simulink model "gm_comm8qamtxrxhdl"  (R2025b)
settings: Solver=FixedStepDiscrete  StartTime=0.0  StopTime=20000*qam_params.symbolPeriod  RelTol=1e-3
PreLoadFcn:
  | qam_params = comm8qamtxrxhdl_init;
InitFcn:
  | qam_params = comm8qamtxrxhdl_init;
undefined symbols (not defined in the file or in its folder): Add, Shift
libraries: simulink x4, hdlsllib x4, dspsigops x2, commchan3 x1, commrflib2 x1, dsphdlmathfun2 x1, dsphdlsigops2 x1, dspmlti4 x1, simulink_need_slupdate x1, hdlmdlgenlib x1, commdigbbndam3 x1, commsequence2 x1
(part 3 of 3)

== system gm_comm8qamtxrxhdl/QAM Tx HDL/Data Generation & Packetization/Group Bits ==
  Bits In : Inport  OutDataTypeStr=boolean  PortDimensions=1  SampleTime=3.33333333333333e-07
  Bit Concat : hdlsllib/Logic and Bit Operations/Bit Concat  numInputs=3
  Delay : Delay  DelayLength=double(1)  InitialCondition=0  SampleTime=3.33333333333333e-07
  Delay4 : Delay  DelayLength=double(2)  InitialCondition=0  SampleTime=3.33333333333333e-07
  Delay5 : Delay  DelayLength=double(1)  InitialCondition=0  SampleTime=3.33333333333333e-07
  Downsample : DownSample  N=double(3)  phase=double(0)  RateOptions=Allow multirate processing  AllowArbitraryFixedInput=on
  Integer Out : Outport  SampleTime=1e-06  VectorParamsAs1DForOutWhenUnconnected=off
  wires:
  Delay/1 -> Downsample/1
  Bits In/1 -> Bit Concat/3, Delay4/1, Delay5/1
  Delay4/1 -> Bit Concat/1
  Downsample/1 -> Integer Out/1
  Delay5/1 -> Bit Concat/2
  Bit Concat/1 -> Delay/1

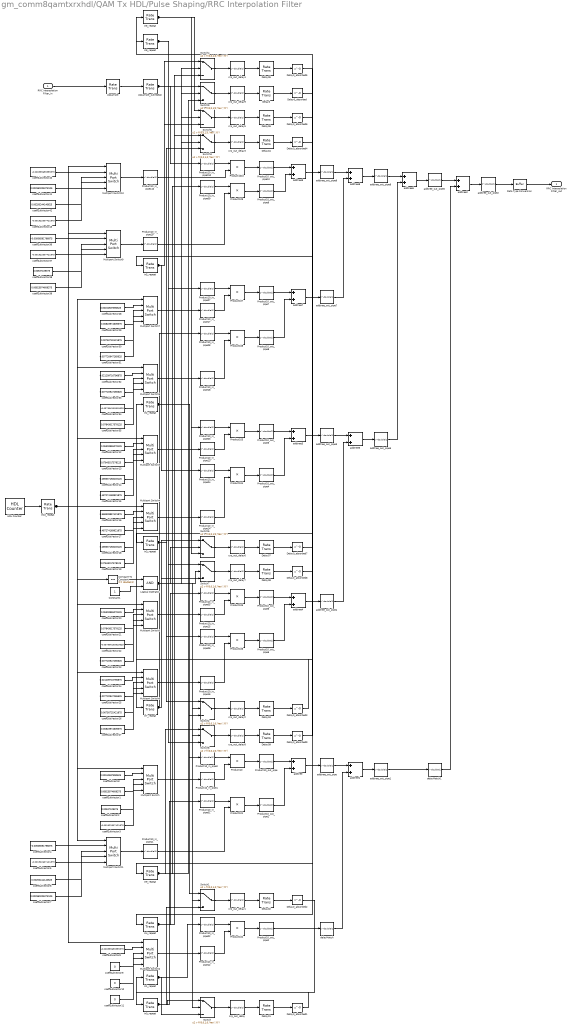
== system gm_comm8qamtxrxhdl/QAM Tx HDL/Pulse Shaping/RRC Interpolation Filter ==
  RRC Interpolation Filter_In : Inport  OutDataTypeStr=fixdt(1, 16, 15)  SampleTime=1e-06
      settings: SignalType=complex
  Compare To Constant : simulink/Logic and Bit Operations/Compare To Constant  relop===  const=double(3)  OutDataTypeStr=boolean
  Constant1 : Constant  OutDataTypeStr=fixdt(0, 1, 0)  SampleTime=8.33333333333333e-08
  Data Type Conversion : hdlmdlgenlib/Buffer
  Delay0 : RateTransition  InitialCondition=double(0)  OutPortSampleTimeOpt=Multiple of input port sample time  OutPortSampleTimeMultiple=3
  Delay01 : RateTransition  InitialCondition=double(0)  OutPortSampleTimeOpt=Multiple of input port sample time  OutPortSampleTimeMultiple=3
  Delay02 : RateTransition  InitialCondition=double(0)  OutPortSampleTimeOpt=Multiple of input port sample time  OutPortSampleTimeMultiple=3
  Delay03 : RateTransition  InitialCondition=double(0)  OutPortSampleTimeOpt=Multiple of input port sample time  OutPortSampleTimeMultiple=3
  Delay04 : RateTransition  InitialCondition=double(0)  OutPortSampleTimeOpt=Multiple of input port sample time  OutPortSampleTimeMultiple=3
  Delay05 : RateTransition  InitialCondition=double(0)  OutPortSampleTimeOpt=Multiple of input port sample time  OutPortSampleTimeMultiple=3
  Delay06 : RateTransition  InitialCondition=double(0)  OutPortSampleTimeOpt=Multiple of input port sample time  OutPortSampleTimeMultiple=3
  Delay07 : RateTransition  InitialCondition=double(0)  OutPortSampleTimeOpt=Multiple of input port sample time  OutPortSampleTimeMultiple=3
  Delay08 : RateTransition  InitialCondition=double(0)  OutPortSampleTimeOpt=Multiple of input port sample time  OutPortSampleTimeMultiple=3
  Delay09 : RateTransition  InitialCondition=double(0)  OutPortSampleTimeOpt=Multiple of input port sample time  OutPortSampleTimeMultiple=3
  Delay0_absorbed{,1..9} (10 alike) : Delay  DelayLength=0
  HDL Counter : hdlsllib/Sources/HDL Counter  CountType=Count limited  CountInit=double(0)  CountStep=double(1)  CountMax=double(3)  CountFromType=Initial value  CountFrom=double(0)  CountResetPort=off  CountLoadPort=off  CountEnbPort=off  CountDirPort=off  CountHitOutputPort=off  CountDataType=Unsigned  CountWordLen=2  CountFracLen=0  CountSampTime=2.5e-07
  Logical Operator : Logic  AllPortsSameDT=off  OutDataTypeStr=fixdt(0, 1, 0)  SampleTime=8.33333333333333e-08
  Multiport Switch{,1..10} (11 alike) : MultiPortSwitch  DataPortOrder=Zero-based contiguous  Inputs=4  DiagnosticForDefault=None  zeroidx=on  OutDataTypeStr=fixdt(1, 16, 15)  SampleTime=8.33333333333333e-08  SaturateOnIntegerOverflow=off  InputSameDT=off
  Product{10,101..109,1010} (11 alike) : Product  Inputs=**  OutDataTypeStr=fixdt(1, 16, 15)  RndMeth=Nearest  SaturateOnIntegerOverflow=on  SampleTime=8.33333333333333e-08
  Product10_in_pipe{0..1,11..19,110} (12 alike) : Delay  DelayLength=double(1)  InitialCondition=0  SampleTime=8.33333333333333e-08
  Product10_in_pipe01 : Delay  DelayLength=double(1)  InitialCondition=0  SampleTime=8.33333333333333e-08
  Product10_in_pipe010 : Delay  DelayLength=double(1)  InitialCondition=0  SampleTime=8.33333333333333e-08
  Product10_in_pipe02 : Delay  DelayLength=double(1)  InitialCondition=0  SampleTime=8.33333333333333e-08
  Product10_in_pipe03 : Delay  DelayLength=double(1)  InitialCondition=0  SampleTime=8.33333333333333e-08
  Product10_in_pipe04 : Delay  DelayLength=double(1)  InitialCondition=0  SampleTime=8.33333333333333e-08
  Product10_in_pipe05 : Delay  DelayLength=double(1)  InitialCondition=0  SampleTime=8.33333333333333e-08
  Product10_in_pipe06 : Delay  DelayLength=double(1)  InitialCondition=0  SampleTime=8.33333333333333e-08
  Product10_in_pipe07 : Delay  DelayLength=double(1)  InitialCondition=0  SampleTime=8.33333333333333e-08
  Product10_in_pipe08 : Delay  DelayLength=double(1)  InitialCondition=0  SampleTime=8.33333333333333e-08
  Product10_in_pipe09 : Delay  DelayLength=double(1)  InitialCondition=0  SampleTime=8.33333333333333e-08
  Product10_out_pipe{,1..10} (11 alike) : Delay  DelayLength=double(2)  InitialCondition=0  SampleTime=8.33333333333333e-08
  Switch{,1..9} (10 alike) : Switch  Criteria=u2 > Threshold  Threshold="fi(0,0,1,0,\"hex\",\"0\")"  OutDataTypeStr=fixdt(1, 16, 15)  SampleTime=8.33333333333333e-08  SaturateOnIntegerOverflow=off  InputSameDT=off
  Upsample : RateTransition  Integrity=off  Deterministic=off  OutPortSampleTimeOpt=Multiple of input port sample time  OutPortSampleTimeMultiple=1/4
  Upsample_outrepeat : RateTransition  Integrity=off  Deterministic=off  OutPortSampleTimeOpt=Multiple of input port sample time  OutPortSampleTimeMultiple=1/3
  addtree{,1..9} (10 alike) : Sum  OutDataTypeStr=fixdt(1, 16, 15)  RndMeth=Nearest  SaturateOnIntegerOverflow=on  SampleTime=8.33333333333333e-08
  addtree_out_pipe{,1..9} (10 alike) : Delay  DelayLength=double(1)  InitialCondition=0  SampleTime=8.33333333333333e-08
  coeffSubVector : Constant  Value=0.00152587890625  OutDataTypeStr=fixdt(1, 16, 15)  SampleTime=8.33333333333333e-08
  coeffSubVector1 : Constant  Value=0.00823974609375  OutDataTypeStr=fixdt(1, 16, 15)  SampleTime=8.33333333333333e-08
  coeffSubVector10 : Constant  Value=0  OutDataTypeStr=fixdt(1, 16, 15)  SampleTime=8.33333333333333e-08
  coeffSubVector11 : Constant  Value=0  OutDataTypeStr=fixdt(1, 16, 15)  SampleTime=8.33333333333333e-08
  coeffSubVector12 : Constant  Value=-0.05303955078125  OutDataTypeStr=fixdt(1, 16, 15)  SampleTime=8.33333333333333e-08
  coeffSubVector13 : Constant  Value=0.07843017578125  OutDataTypeStr=fixdt(1, 16, 15)  SampleTime=8.33333333333333e-08
  coeffSubVector14 : Constant  Value=0.289337158203125  OutDataTypeStr=fixdt(1, 16, 15)  SampleTime=8.33333333333333e-08
  coeffSubVector15 : Constant  Value=0.487274169921875  OutDataTypeStr=fixdt(1, 16, 15)  SampleTime=8.33333333333333e-08
  coeffSubVector16 : Constant  Value=0.568328857421875  OutDataTypeStr=fixdt(1, 16, 15)  SampleTime=8.33333333333333e-08
  coeffSubVector17 : Constant  Value=0.487274169921875  OutDataTypeStr=fixdt(1, 16, 15)  SampleTime=8.33333333333333e-08
  coeffSubVector18 : Constant  Value=0.289337158203125  OutDataTypeStr=fixdt(1, 16, 15)  SampleTime=8.33333333333333e-08
  coeffSubVector19 : Constant  Value=0.07843017578125  OutDataTypeStr=fixdt(1, 16, 15)  SampleTime=8.33333333333333e-08
  coeffSubVector2 : Constant  Value=0.00537109375  OutDataTypeStr=fixdt(1, 16, 15)  SampleTime=8.33333333333333e-08
  coeffSubVector20 : Constant  Value=-0.05303955078125  OutDataTypeStr=fixdt(1, 16, 15)  SampleTime=8.33333333333333e-08
  coeffSubVector21 : Constant  Value=-0.07843017578125  OutDataTypeStr=fixdt(1, 16, 15)  SampleTime=8.33333333333333e-08
  coeffSubVector22 : Constant  Value=-0.037506103515625  OutDataTypeStr=fixdt(1, 16, 15)  SampleTime=8.33333333333333e-08
  coeffSubVector{23,25,31,33} (4 alike) : Constant  Value=0.007720947265625  OutDataTypeStr=fixdt(1, 16, 15)  SampleTime=8.33333333333333e-08
  coeffSubVector24 : Constant  Value=0.021209716796875  OutDataTypeStr=fixdt(1, 16, 15)  SampleTime=8.33333333333333e-08
  coeffSubVector26 : Constant  Value=-0.00750732421875  OutDataTypeStr=fixdt(1, 16, 15)  SampleTime=8.33333333333333e-08
  coeffSubVector27 : Constant  Value=-0.00823974609375  OutDataTypeStr=fixdt(1, 16, 15)  SampleTime=8.33333333333333e-08
  coeffSubVector28 : Constant  Value=0.00152587890625  OutDataTypeStr=fixdt(1, 16, 15)  SampleTime=8.33333333333333e-08
  coeffSubVector29 : Constant  Value=-0.00823974609375  OutDataTypeStr=fixdt(1, 16, 15)  SampleTime=8.33333333333333e-08
  coeffSubVector{3,5,37,43} (4 alike) : Constant  Value=-0.001922607421875  OutDataTypeStr=fixdt(1, 16, 15)  SampleTime=8.33333333333333e-08
  coeffSubVector30 : Constant  Value=-0.00750732421875  OutDataTypeStr=fixdt(1, 16, 15)  SampleTime=8.33333333333333e-08
  coeffSubVector32 : Constant  Value=0.021209716796875  OutDataTypeStr=fixdt(1, 16, 15)  SampleTime=8.33333333333333e-08
  coeffSubVector34 : Constant  Value=-0.037506103515625  OutDataTypeStr=fixdt(1, 16, 15)  SampleTime=8.33333333333333e-08
  coeffSubVector35 : Constant  Value=-0.07843017578125  OutDataTypeStr=fixdt(1, 16, 15)  SampleTime=8.33333333333333e-08
  coeffSubVector36 : Constant  Value=-0.00506591796875  OutDataTypeStr=fixdt(1, 16, 15)  SampleTime=8.33333333333333e-08
  coeffSubVector38 : Constant  Value=0.00537109375  OutDataTypeStr=fixdt(1, 16, 15)  SampleTime=8.33333333333333e-08
  coeffSubVector39 : Constant  Value=0.00823974609375  OutDataTypeStr=fixdt(1, 16, 15)  SampleTime=8.33333333333333e-08
  coeffSubVector4 : Constant  Value=-0.00506591796875  OutDataTypeStr=fixdt(1, 16, 15)  SampleTime=8.33333333333333e-08
  coeffSubVector40 : Constant  Value=-0.000335693359375  OutDataTypeStr=fixdt(1, 16, 15)  SampleTime=8.33333333333333e-08
  coeffSubVector41 : Constant  Value=0.002960205078125  OutDataTypeStr=fixdt(1, 16, 15)  SampleTime=8.33333333333333e-08
  coeffSubVector42 : Constant  Value=0.00250244140625  OutDataTypeStr=fixdt(1, 16, 15)  SampleTime=8.33333333333333e-08
  coeffSubVector6 : Constant  Value=0.00250244140625  OutDataTypeStr=fixdt(1, 16, 15)  SampleTime=8.33333333333333e-08
  coeffSubVector7 : Constant  Value=0.002960205078125  OutDataTypeStr=fixdt(1, 16, 15)  SampleTime=8.33333333333333e-08
  coeffSubVector8 : Constant  Value=-0.000335693359375  OutDataTypeStr=fixdt(1, 16, 15)  SampleTime=8.33333333333333e-08
  coeffSubVector9 : Constant  Value=0  OutDataTypeStr=fixdt(1, 16, 15)  SampleTime=8.33333333333333e-08
  crp_out_delay{,1..9} (10 alike) : Delay  DelayLength=double(1)  InitialCondition=0  SampleTime=8.33333333333333e-08
  delayMatch : Delay  DelayLength=double(1)  InitialCondition=0  SampleTime=8.33333333333333e-08
  delayMatch1 : Delay  DelayLength=double(1)  InitialCondition=0  SampleTime=8.33333333333333e-08
  in0_repeat : RateTransition  Integrity=off  Deterministic=off  OutPortSampleTimeOpt=Multiple of input port sample time  OutPortSampleTimeMultiple=1/3
  in10_repeat : RateTransition  Integrity=off  Deterministic=off  OutPortSampleTimeOpt=Multiple of input port sample time  OutPortSampleTimeMultiple=1/3
  in1_repeat : RateTransition  Integrity=off  Deterministic=off  OutPortSampleTimeOpt=Multiple of input port sample time  OutPortSampleTimeMultiple=1/3
  in2_repeat : RateTransition  Integrity=off  Deterministic=off  OutPortSampleTimeOpt=Multiple of input port sample time  OutPortSampleTimeMultiple=1/3
  in3_repeat : RateTransition  Integrity=off  Deterministic=off  OutPortSampleTimeOpt=Multiple of input port sample time  OutPortSampleTimeMultiple=1/3
  in4_repeat : RateTransition  Integrity=off  Deterministic=off  OutPortSampleTimeOpt=Multiple of input port sample time  OutPortSampleTimeMultiple=1/3
  in5_repeat : RateTransition  Integrity=off  Deterministic=off  OutPortSampleTimeOpt=Multiple of input port sample time  OutPortSampleTimeMultiple=1/3
  in6_repeat : RateTransition  Integrity=off  Deterministic=off  OutPortSampleTimeOpt=Multiple of input port sample time  OutPortSampleTimeMultiple=1/3
  in7_repeat : RateTransition  Integrity=off  Deterministic=off  OutPortSampleTimeOpt=Multiple of input port sample time  OutPortSampleTimeMultiple=1/3
  in8_repeat : RateTransition  Integrity=off  Deterministic=off  OutPortSampleTimeOpt=Multiple of input port sample time  OutPortSampleTimeMultiple=1/3
  in9_repeat : RateTransition  Integrity=off  Deterministic=off  OutPortSampleTimeOpt=Multiple of input port sample time  OutPortSampleTimeMultiple=1/3
  RRC Interpolation Filter_out : Outport  OutDataTypeStr=fixdt(1, 16, 15)  SampleTime=8.33333333333333e-08
      settings: SignalType=complex
  wires:
  addtree_out_pipe1/1 -> delayMatch1/1
  coeffSubVector2/1 -> Multiport Switch/4
  Product10_in_pipe08/1 -> Product108/1
  addtree2/1 -> addtree_out_pipe2/1
  Switch/1 -> crp_out_delay/1
  addtree8/1 -> addtree_out_pipe8/1
  addtree_out_pipe9/1 -> addtree8/1
  Logical Operator/1 -> Switch/2, Switch1/2, Switch2/2, Switch4/2, Switch5/2, Switch6/2, Switch7/2, Switch9/2, Switch3/2, Switch8/2
  Product10_in_pipe010/1 -> Product1010/1
  addtree/1 -> addtree_out_pipe/1
  Product10_out_pipe3/1 -> addtree3/1
  addtree5/1 -> addtree_out_pipe5/1
  Delay09/1 -> Delay0_absorbed9/1
  Product10_in_pipe09/1 -> Product109/1
  Product10_in_pipe01/1 -> Product101/1
  coeffSubVector27/1 -> Multiport Switch6/5
  Product10_in_pipe18/1 -> Product108/2
  coeffSubVector24/1 -> Multiport Switch6/2
  Product10_in_pipe17/1 -> Product107/2
  addtree_out_pipe4/1 -> addtree5/2
  Multiport Switch9/1 -> Product10_in_pipe19/1
  Delay0_absorbed/1 -> in9_repeat/1
  Product108/1 -> Product10_out_pipe8/1
  addtree_out_pipe7/1 -> addtree8/2
  Product10_in_pipe07/1 -> Product107/1
  Delay0_absorbed1/1 -> in1_repeat/1
  coeffSubVector36/1 -> Multiport Switch9/2
  Product10_in_pipe16/1 -> Product106/2
  Product10_in_pipe03/1 -> Product103/1
  coeffSubVector40/1 -> Multiport Switch10/2
  Upsample/1 -> Upsample_outrepeat/1
  Multiport Switch4/1 -> Product10_in_pipe14/1
  Product10_in_pipe12/1 -> Product102/2
  addtree9/1 -> addtree_out_pipe9/1
  coeffSubVector21/1 -> Multiport Switch5/3
  Product10_in_pipe05/1 -> Product105/1
  Switch7/1 -> crp_out_delay7/1
  Multiport Switch10/1 -> Product10_in_pipe110/1
  Product1010/1 -> Product10_out_pipe10/1
  Product10_in_pipe06/1 -> Product106/1
  coeffSubVector37/1 -> Multiport Switch9/3
  Product10_in_pipe15/1 -> Product105/2
  Product109/1 -> Product10_out_pipe9/1
  Product10_in_pipe02/1 -> Product102/1
  Product10_in_pipe14/1 -> Product104/2
  Product101/1 -> Product10_out_pipe1/1
  in4_repeat/1 -> Switch4/3, Switch3/1, Product10_in_pipe05/1
  Product107/1 -> Product10_out_pipe7/1
  coeffSubVector43/1 -> Multiport Switch10/5
  Product10_in_pipe04/1 -> Product104/1
  Product10_in_pipe0/1 -> Product10/1
  Delay06/1 -> Delay0_absorbed6/1
  coeffSubVector38/1 -> Multiport Switch9/4
  Product104/1 -> Product10_out_pipe4/1
  Product10_in_pipe13/1 -> Product103/2
  Product10_out_pipe7/1 -> addtree7/1
  addtree1/1 -> addtree_out_pipe1/1
  addtree4/1 -> addtree_out_pipe4/1
  coeffSubVector8/1 -> Multiport Switch2/2
  coeffSubVector13/1 -> Multiport Switch3/3
  addtree_out_pipe8/1 -> addtree6/1
  Constant1/1 -> Logical Operator/2
  Product10/1 -> Product10_out_pipe/1
  coeffSubVector16/1 -> Multiport Switch4/2
  Product10_in_pipe1/1 -> Product10/2
  Product10_out_pipe9/1 -> addtree9/2
  Product103/1 -> Product10_out_pipe3/1
  addtree_out_pipe5/1 -> addtree6/2
  Product10_out_pipe8/1 -> addtree7/2
  addtree7/1 -> addtree_out_pipe7/1
  crp_out_delay3/1 -> Delay04/1
  addtree6/1 -> addtree_out_pipe6/1
  Switch5/1 -> crp_out_delay5/1
  coeffSubVector41/1 -> Multiport Switch10/3
  Multiport Switch7/1 -> Product10_in_pipe17/1
  in10_repeat/1 -> Multiport Switch6/1, Multiport Switch/1, Multiport Switch8/1, Multiport Switch4/1, Multiport Switch2/1, Compare To Constant/1, Multiport Switch10/1, Multiport Switch1/1, Multiport Switch5/1, Multiport Switch9/1, Multiport Switch3/1, Multiport Switch7/1
  Product106/1 -> Product10_out_pipe6/1
  addtree_out_pipe6/1 -> addtree2/1
  Product102/1 -> Product10_out_pipe2/1
  Product105/1 -> Product10_out_pipe5/1
  addtree3/1 -> addtree_out_pipe3/1
  Compare To Constant/1 -> Logical Operator/1
  Switch9/1 -> crp_out_delay9/1
  Product10_out_pipe10/1 -> addtree9/1
  coeffSubVector42/1 -> Multiport Switch10/4
  Switch1/1 -> crp_out_delay1/1
  coeffSubVector39/1 -> Multiport Switch9/5
  Multiport Switch8/1 -> Product10_in_pipe18/1
  coeffSubVector35/1 -> Multiport Switch8/5
  coeffSubVector34/1 -> Multiport Switch8/4
  coeffSubVector33/1 -> Multiport Switch8/3
  coeffSubVector32/1 -> Multiport Switch8/2
  coeffSubVector31/1 -> Multiport Switch7/5
  coeffSubVector30/1 -> Multiport Switch7/4
  coeffSubVector29/1 -> Multiport Switch7/3
  coeffSubVector28/1 -> Multiport Switch7/2
  Product10_out_pipe6/1 -> addtree4/2
  Product10_in_pipe19/1 -> Product109/2
  Multiport Switch6/1 -> Product10_in_pipe16/1
  coeffSubVector26/1 -> Multiport Switch6/4
  coeffSubVector25/1 -> Multiport Switch6/3
  Product10_out_pipe4/1 -> addtree3/2
  Delay0/1 -> Delay0_absorbed/1
  Product10_out_pipe5/1 -> addtree4/1
  Multiport Switch5/1 -> Product10_in_pipe15/1
  coeffSubVector23/1 -> Multiport Switch5/5
  coeffSubVector22/1 -> Multiport Switch5/4
  coeffSubVector20/1 -> Multiport Switch5/2
  coeffSubVector10/1 -> Multiport Switch2/4
  addtree_out_pipe3/1 -> addtree5/1
  Product10_in_pipe11/1 -> Product101/2
  coeffSubVector19/1 -> Multiport Switch4/5
  Delay04/1 -> Delay0_absorbed4/1
  Multiport Switch1/1 -> Product10_in_pipe11/1
  coeffSubVector18/1 -> Multiport Switch4/4
  coeffSubVector17/1 -> Multiport Switch4/3
  Multiport Switch3/1 -> Product10_in_pipe13/1
  coeffSubVector15/1 -> Multiport Switch3/5
  coeffSubVector14/1 -> Multiport Switch3/4
  Delay05/1 -> Delay0_absorbed5/1
  Switch4/1 -> crp_out_delay4/1
  in2_repeat/1 -> Product10_in_pipe0/1, Switch1/1, Switch2/3
  coeffSubVector12/1 -> Multiport Switch3/2
  addtree_out_pipe2/1 -> Data Type Conversion/1
  delayMatch1/1 -> addtree2/2
  delayMatch/1 -> addtree1/2
  Multiport Switch2/1 -> Product10_in_pipe12/1
  coeffSubVector11/1 -> Multiport Switch2/5
  in6_repeat/1 -> Switch6/3, Switch5/1, Product10_in_pipe03/1
  coeffSubVector9/1 -> Multiport Switch2/3
  addtree_out_pipe/1 -> addtree1/1
  coeffSubVector6/1 -> Multiport Switch1/4
  Product10_out_pipe1/1 -> addtree/2
  Delay0_absorbed6/1 -> in5_repeat/1
  coeffSubVector7/1 -> Multiport Switch1/5
  coeffSubVector5/1 -> Multiport Switch1/3
  coeffSubVector4/1 -> Multiport Switch1/2
  Product10_out_pipe/1 -> addtree/1
  Multiport Switch/1 -> Product10_in_pipe1/1
  Switch3/1 -> crp_out_delay3/1
  coeffSubVector3/1 -> Multiport Switch/5
  coeffSubVector1/1 -> Multiport Switch/3
  coeffSubVector/1 -> Multiport Switch/2
  Switch8/1 -> crp_out_delay8/1
  in1_repeat/1 -> Product10_in_pipe02/1, Switch/3
  Delay0_absorbed5/1 -> in4_repeat/1
  Switch6/1 -> crp_out_delay6/1
  Delay02/1 -> Delay0_absorbed2/1
  Switch2/1 -> crp_out_delay2/1
  Delay0_absorbed9/1 -> in8_repeat/1
  crp_out_delay9/1 -> Delay0/1
  Delay07/1 -> Delay0_absorbed7/1
  Delay08/1 -> Delay0_absorbed8/1
  in0_repeat/1 -> Product10_in_pipe01/1, Switch/1, Switch1/3
  Delay03/1 -> Delay0_absorbed3/1
  in7_repeat/1 -> Switch6/1, Product10_in_pipe08/1, Switch7/3
  Delay01/1 -> Delay0_absorbed1/1
  crp_out_delay2/1 -> Delay03/1
  crp_out_delay8/1 -> Delay09/1
  crp_out_delay7/1 -> Delay08/1
  crp_out_delay/1 -> Delay01/1
  crp_out_delay6/1 -> Delay07/1
  crp_out_delay5/1 -> Delay06/1
  crp_out_delay4/1 -> Delay05/1
  crp_out_delay1/1 -> Delay02/1
  Data Type Conversion/1 -> RRC Interpolation Filter_out/1
  HDL Counter/1 -> in10_repeat/1
  RRC Interpolation Filter_In/1 -> Upsample/1
  in9_repeat/1 -> Product10_in_pipe09/1, Switch9/3, Switch8/1
  in8_repeat/1 -> Product10_in_pipe07/1, Switch8/3, Switch7/1
  in5_repeat/1 -> Product10_in_pipe04/1, Switch5/3, Switch4/1
  in3_repeat/1 -> Product10_in_pipe06/1, Switch3/3, Switch2/1
  Upsample_outrepeat/1 -> Product10_in_pipe010/1, Switch9/1
  Product10_in_pipe110/1 -> Product1010/2
  Product10_out_pipe2/1 -> delayMatch/1
  Delay0_absorbed2/1 -> in0_repeat/1
  Delay0_absorbed7/1 -> in6_repeat/1
  Delay0_absorbed4/1 -> in3_repeat/1
  Delay0_absorbed3/1 -> in2_repeat/1
  Delay0_absorbed8/1 -> in7_repeat/1

== system gm_comm8qamtxrxhdl/QAM Rx HDL/Coarse Frequency Offset Correction/Frequency Offset Estimation/Enabled Wire ==
  In1 : Inport
  Enable : EnablePort
  Out1 : Outport  InitialOutput=0  VectorParamsAs1DForOutWhenUnconnected=off
  wires:
  In1/1 -> Out1/1

== system gm_comm8qamtxrxhdl/QAM Rx HDL/Coarse Frequency Offset Correction/Frequency Offset Estimation/Raise to Power 4 ==
  In1 : Inport
  Delay1 : Delay  InitialCondition=0
  Delay4 : Delay  DelayLength=4  InitialCondition=0
  Delay5 : Delay  DelayLength=4  InitialCondition=0
  Product : Product  OutDataTypeStr=fixdt(1,16,15)
  Product1 : Product  OutDataTypeStr=fixdt(1,16,15)
  Out1 : Outport  VectorParamsAs1DForOutWhenUnconnected=off
  wires:
  Delay1/1 -> Product/1, Product/2
  In1/1 -> Delay1/1
  Delay4/1 -> Product1/1, Product1/2
  Delay5/1 -> Out1/1
  Product1/1 -> Delay5/1
  Product/1 -> Delay4/1

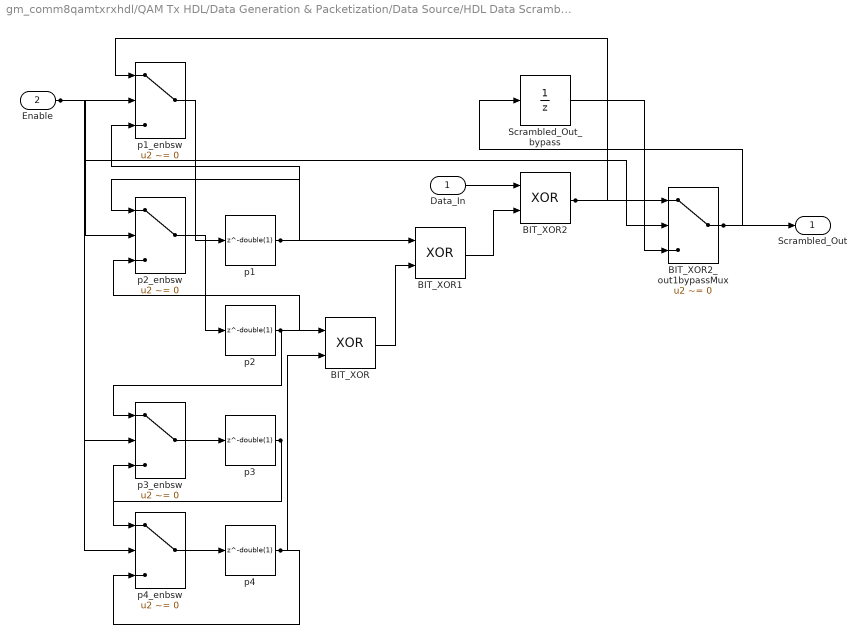
== system gm_comm8qamtxrxhdl/QAM Tx HDL/Data Generation & Packetization/Data Source/HDL Data Scrambler ==
  Data_In : Inport  OutDataTypeStr=boolean  PortDimensions=1  SampleTime=3.33333333333333e-07
  Enable : Inport  Port=2  OutDataTypeStr=boolean  SampleTime=3.33333333333333e-07
  BIT_XOR : Logic  Operator=XOR  AllPortsSameDT=off  OutDataTypeStr=boolean  SampleTime=3.33333333333333e-07
  BIT_XOR1 : Logic  Operator=XOR  AllPortsSameDT=off  OutDataTypeStr=boolean  SampleTime=3.33333333333333e-07
  BIT_XOR2 : Logic  Operator=XOR  AllPortsSameDT=off  OutDataTypeStr=boolean  SampleTime=3.33333333333333e-07
  BIT_XOR2_out1bypassMux : Switch  Criteria=u2 ~= 0  Threshold=double(0)  OutDataTypeStr=boolean  SampleTime=3.33333333333333e-07  SaturateOnIntegerOverflow=off  InputSameDT=off
  Scrambled_Out_bypass : UnitDelay  SampleTime=3.33333333333333e-07
  p{1..4} (4 alike) : Delay  DelayLength=double(1)  InitialCondition=0
  p1_enbsw : Switch  Criteria=u2 ~= 0  Threshold=double(0)  OutDataTypeStr=boolean  SampleTime=3.33333333333333e-07  SaturateOnIntegerOverflow=off  InputSameDT=off
  p2_enbsw : Switch  Criteria=u2 ~= 0  Threshold=double(0)  OutDataTypeStr=boolean  SampleTime=3.33333333333333e-07  SaturateOnIntegerOverflow=off  InputSameDT=off
  p3_enbsw : Switch  Criteria=u2 ~= 0  Threshold=double(0)  OutDataTypeStr=boolean  SampleTime=3.33333333333333e-07  SaturateOnIntegerOverflow=off  InputSameDT=off
  p4_enbsw : Switch  Criteria=u2 ~= 0  Threshold=double(0)  OutDataTypeStr=boolean  SampleTime=3.33333333333333e-07  SaturateOnIntegerOverflow=off  InputSameDT=off
  Scrambled_Out : Outport  SampleTime=3.33333333333333e-07  InitialOutput=0  VectorParamsAs1DForOutWhenUnconnected=off
  wires:
  p1/1 -> p2_enbsw/1, p1_enbsw/3, BIT_XOR1/1
  Enable/1 -> p3_enbsw/2, p1_enbsw/2, p2_enbsw/2, p4_enbsw/2, BIT_XOR2_out1bypassMux/2
  p4_enbsw/1 -> p4/1
  p1_enbsw/1 -> p1/1
  p2_enbsw/1 -> p2/1
  p3_enbsw/1 -> p3/1
  p2/1 -> p2_enbsw/3, p3_enbsw/1, BIT_XOR/1
  p3/1 -> p4_enbsw/1, p3_enbsw/3
  p4/1 -> p4_enbsw/3, BIT_XOR/2
  BIT_XOR/1 -> BIT_XOR1/2
  Data_In/1 -> BIT_XOR2/1
  BIT_XOR1/1 -> BIT_XOR2/2
  Scrambled_Out_bypass/1 -> BIT_XOR2_out1bypassMux/3
  BIT_XOR2/1 -> p1_enbsw/1, BIT_XOR2_out1bypassMux/1
  BIT_XOR2_out1bypassMux/1 -> Scrambled_Out_bypass/1, Scrambled_Out/1

== matlab function gm_comm8qamtxrxhdl/QAM Rx HDL/Timing Recovery/Interpolation Control ==
  data: Delta input; Underflow output; mu output
function [Underflow, mu] = Interpolation_ctrl(Delta)
% Implementation of modulo-1 counter for interpolation control listed in
% Figure 8.4.19 of "Digital Communications - A Discrete-Time Approach"
% by Michael Rice. See design details in Chapter 8.4.3 of the same book.
% 
% Input:
%   Delta - Loop filter output. If loop is in lock, delta would be small
% Output:
%   Underflow - Indicator of counter underflow. This is the strobe signal
%               for downstream processing
%   mu - Difference between actual sampling instant and the optimal instant,
%        between zero and one
%#codegen

% delay1 - Counter value delayed by 1 sample
% Regtemp - The estimated timing error normalized by half QPSK symbols

W = 16; % accumulator wordlength
F = 15; % accumulator fraction length

persistent delay1 Regtemp;  
if isempty(delay1)
    delay1  = fi(0,1,W,F);
    Regtemp = fi(0,1,W,F);
end

mask = fi(1-2^(-F),1,W,F);

counter = bitand(mask,delay1)-Delta-fi(0.5,1,W,F); % decrementing counter
% if delay1 is a nonnegative number,
% then mod(delay1,1) equals the fractional part of delay1

if counter < 0
    Underflow = true;
    Regtemp = bitshift(bitand(mask,delay1),1);     
else
    Underflow = false;
end

mu = Regtemp;

% Update delay buffer
% delay1 = counter;
if counter<0
    delay1 = fi(counter+1,1,W,F); %make sure delay1 is nonnegative
else
    delay1 = fi(counter,1,W,F);
end

== matlab function gm_comm8qamtxrxhdl/QAM Rx HDL/Timing Recovery/Timing Error Detector ==
  data: In input; strobe input; e output
function e = TED(In, strobe)
% Zero-Crossing Timing Error Detector. See "Zero-Crossing Timing Error
% Detector" section in Chapter 8.4.1 of "Digital Communications - A
% Discrete-Time Approach" by Michael Rice. For bit stuffing/stripping
% details, see page 490-494 of the same book.
%
% Input: 
%   In - Input samples, interpolation result
%   strobe - Signal to enable timing error calculation
% Output:
%   e - Timing error
%#codegen

persistent delay1_R delay1_I delay2_R delay2_I delayStrobe; 
% Input delayed by one and 2 samples, and
% Enable signal delayed by one sample
if isempty(delay1_R)    
    delay1_R=fi(0,1,16,15);
    delay1_I=fi(0,1,16,15);
    delay2_R=fi(0,1,16,15);
    delay2_I=fi(0,1,16,15);    
    delayStrobe = false;
end

In_Real = real(In);
In_Imag = imag(In);

if strobe==true && delayStrobe~=strobe
    if ( bitget(delay2_R,16)==bitget(In_Real,16) )         
        OP1=fi(0,1,16,15);
    elseif bitget(delay2_R,16)==true         
        OP1=fi(-1*bitshift(delay1_R,1),1,16,15);
    else        
        OP1=fi(bitshift(delay1_R,1),1,16,15);
    end
    
    if ( bitget(delay2_I,16)==bitget(In_Imag,16) )        
        OP2=fi(0,1,16,15);
    elseif bitget(delay2_I,16)==true        
        OP2=fi(-1*bitshift(delay1_I,1),1,16,15);
    else        
        OP2=fi(bitshift(delay1_I,1),1,16,15);
    end
else
    OP1=fi(0,1,16,15);
    OP2=fi(0,1,16,15);
end

e = fi(OP1+OP2,1,16,15);


if delayStrobe~=strobe
    % Shift contents in delay register
    delay2_R = delay1_R;
    delay1_R = In_Real;
    delay2_I = delay1_I;
    delay1_I = In_Imag;
elseif strobe==true
    % Two consecutive high strobes
    delay2_R = fi(0,1,16,15); % Stuff missing sample
    delay1_R = In_Real; 
    delay2_I = fi(0,1,16,15); % Stuff missing sample
    delay1_I = In_Imag; 
end

% If both current and previous enable signals are 0, skip current sample
% and keep the delayed signals unchanged. (Bit stripping)
delayStrobe = strobe;

== matlab function gm_comm8qamtxrxhdl/QAM Rx HDL/Demodulate/Rectangular QAM Demodulator Baseband ==
  data: u input; y output
function y = Rect8QAMDemod(u)
%#codegen
% HDL-compatible Gray-coded 8-QAM Hard-Decision Demodulator (MinDist = 2)
% Constellation points: I in {-3, -1, +1, +3}, Q in {-1, +1}
I = real(u);
Q = imag(u);
b1 = (I >= 0);       % MSB: 0 for I < 0, 1 for I >= 0
b2 = (abs(I) <= 2);  % Mid: 0 for |I| > 2 (+-3), 1 for |I| <= 2 (+-1)
b3 = (Q < 0);        % LSB: 0 for Q >= 0 (+1), 1 for Q < 0 (-1)
y  = [b1; b2; b3];

== matlab function gm_comm8qamtxrxhdl/QAM Tx HDL/Data Generation & Packetization/Controller FSM/Controller FSM ==
  data: reset_preamble output; load_preamble output; load_data output
function [reset_preamble,load_preamble, load_data] = ControllerFSM()
%#codegen

persistent packState;
persistent stateCounter;

sType = numerictype(0,1,0);
cType = numerictype(0,8,0);

if isempty(packState)
    packState = fi(0,'numerictype',sType);
    stateCounter  = fi(0,'numerictype',cType);
end

Pack_Preamble = fi(0,'numerictype',sType);
Append_Data   = fi(1,'numerictype',sType);

switch(packState)
    case Pack_Preamble  %% Pack_Preamble
        load_preamble  = true;
        reset_preamble = false;
        load_data      = false;
        
        if stateCounter == 41;  %% Pack_Preamble complete
            packState(:) = 1;                   %% move to Append_Data state
            stateCounter(:) = 0;                %% reset counter
        else
            packState(:) = 0;                   %% remain in Pack_Preamble state
            stateCounter(:) = stateCounter +1;  %% increment preamble count
        end
        
    case Append_Data    %% Append_Data
        load_preamble  = false;
        reset_preamble = true;
        load_data      = true;
        
        if stateCounter == 125  %% Append_Data complete
            packState(:) = 0;                   %% move to Pack_Preamble state
            stateCounter(:) = 0;                %% reset counter
        else
            packState(:) = 1;                   %% remain in Append_Data state
            stateCounter(:) = stateCounter +1;  %% increment data count
        end
        
    otherwise
        load_preamble  = false;
        reset_preamble = false;
        load_data      = false;
        stateCounter(:) = 0;
end

== matlab function gm_comm8qamtxrxhdl/Text Message Decoding/  ==
  data: newPacket input; dValid input; RxGo output; framed_data output; bit1 input; bit2 input; bit3 input
function [RxGo,framed_data] = dataframer(newPacket, dValid, bit1, bit2, bit3)
%#codegen

persistent gooddata_so_far frame_index

if isempty(gooddata_so_far)
    gooddata_so_far = false(168,1);
    frame_index = 1;
end

RxGo = false;
framed_data = false(168,1);

if dValid==true
    gooddata_so_far(frame_index:frame_index+2) = [bit1 bit2 bit3];
    frame_index = frame_index+3;
    if (frame_index==169) || (newPacket==true)
        RxGo = true;
        framed_data = gooddata_so_far;
        frame_index = 1;
    end
end

== matlab function gm_comm8qamtxrxhdl/QAM Rx HDL/Magnitude & Phase Recovery/MATLAB Function3 ==
  data: dvalid output; enable input; isPreamble output
function [dvalid,isPreamble] = fcn(enable)
%#codegen

persistent state;
persistent counter;


if isempty(state);
    state      = false;
    counter    = uint8(0);
end


if counter > 42
    isPreamble = true;
else
    isPreamble = false;
end


if state==false
    dvalid=false;
else %state==true
    dvalid=true;
    counter = counter-1;
end


% state transition
if state==false && enable==true
    state=true;
    counter=uint8(56);
elseif state==true && counter==0
    if enable==true % packages come back-to-back
        state      = true;
        counter    = uint8(56);
    else
        state = false;    
    end
end

== matlab function gm_comm8qamtxrxhdl/Text Message Decoding/Descramble and Print/BitsToDecimal1 ==
  data: u input
function BitsToASCII(u)
% Convert bits to ASCII message (8-QAM Option A: 18 chars = 126 bits).

persistent package_counter;
persistent error_counter;
if isempty(package_counter)
    package_counter = 0;
    error_counter   = 0;
end

coder.extrinsic('disp')
coder.extrinsic('num2str')

aa = de2bi(int8('Hello! ~8-QAM~ 0'),7,'left-msb');
bits_ref = double(reshape(aa.',1,[]));
bits_ref = bits_ref(:);

error_counter   = error_counter   + sum(abs(bits_ref - u(1:112)));
package_counter = package_counter + 1;

% Convert binary-valued column vector to 7-bit decimal values.
w = [64 32 16 8 4 2 1]; % binary digit weighting
Nbits = numel(u);
Ny = Nbits/7;
y = zeros(1,Ny);
for i = 0:Ny-1
    y(i+1) = w*u(7*i+(1:7));
end

% Display ASCII message to command window
if rem(package_counter,50)==0
    disp([char(y) '    ==>    BER = ' num2str(error_counter/50/7/16)]);
    error_counter = 0;
else
    disp(char(y));
end
